simulink library "casper_library_sources"  (R2021a)
settings: Solver=ode45  StartTime=0.0  StopTime=10.0  RelTol=1e-3
values from neighbouring files (symbols this model uses):
  a = [lenba, lenpa, lenta]    [bus_addsub_init.m]    (also in bus_logical_init.m; bus_maddsub_init.m; bus_mult_init.m; bus_relational_init.m)
  b = [lenbb, lenpb, lentb]    [bus_addsub_init.m]    (also in bus_logical_init.m; bus_maddsub_init.m; bus_mult_init.m; bus_relational_init.m)
libraries: xbsIndex_r4 x11172, $bdroot x2
(part 6 of 29)

== system casper_library_sources/Correlation Control Block/corr_ctrl_blk/NS 27bit/lfsr_11 ==
  " reset" : Inport
  Assert{1..31} (31 alike) : xbsIndex_r4/Assert  assert_type=on  type_source=Explicitly  gui_display_data_type=Fixed-point  arith_type=Unsigned  n_bits=1  bin_pt=0  preci_type=Single  exp_width=8  frac_width=24  assert_rate=on  rate_source=Explicitly  period=1  output_port=on  block_type=assert
      settings: infoedit=Asserts a user-defined sample rate and/or type on a signal.<P><P>Hardware notes: In hardware this block costs nothing.  block_version=10.1.3
  Concat : xbsIndex_r4/Concat  num_inputs=4  dbl_ovrd=off  block_type=concat
      settings: block_version=10.1.3
  Expression{,1..11} (12 alike) : xbsIndex_r4/Expression  expression=a ^ b  align_bp=on  en=off  latency=0  precision=Full  arith_type=Unsigned  n_bits=8  bin_pt=2  dbl_ovrd=off  block_type=expr
      settings: xl_area=[0, 0, 0, 0, 0, 0, 0]  block_version=10.1.3
  Register1 : xbsIndex_r4/Register  init=seed(3)  rst=on  en=off  dbl_ovrd=off  block_type=register
      settings: xl_area=[0, 0, 0, 0, 0, 0, 0]
  Register10 : xbsIndex_r4/Register  init=seed(11)  rst=on  en=off  dbl_ovrd=off  block_type=register
      settings: xl_area=[0, 0, 0, 0, 0, 0, 0]
  Register11 : xbsIndex_r4/Register  init=seed(12)  rst=on  en=off  dbl_ovrd=off  block_type=register
      settings: xl_area=[0, 0, 0, 0, 0, 0, 0]
  Register12 : xbsIndex_r4/Register  init=seed(13)  rst=on  en=off  dbl_ovrd=off  block_type=register
      settings: xl_area=[0, 0, 0, 0, 0, 0, 0]
  Register13 : xbsIndex_r4/Register  init=seed(14)  rst=on  en=off  dbl_ovrd=off  block_type=register
      settings: xl_area=[0, 0, 0, 0, 0, 0, 0]
  Register14 : xbsIndex_r4/Register  init=seed(15)  rst=on  en=off  dbl_ovrd=off  block_type=register
      settings: xl_area=[0, 0, 0, 0, 0, 0, 0]
  Register15 : xbsIndex_r4/Register  init=seed(16)  rst=on  en=off  dbl_ovrd=off  block_type=register
      settings: xl_area=[0, 0, 0, 0, 0, 0, 0]
  Register16 : xbsIndex_r4/Register  init=seed(17)  rst=on  en=off  dbl_ovrd=off  block_type=register
      settings: xl_area=[0, 0, 0, 0, 0, 0, 0]
  Register{17,19..27} (10 alike) : xbsIndex_r4/Register  init=seed(18)  rst=on  en=off  dbl_ovrd=off  block_type=register
      settings: xl_area=[0, 0, 0, 0, 0, 0, 0]
  Register18 : xbsIndex_r4/Register  init=seed(1)  rst=on  en=off  dbl_ovrd=off  block_type=register
      settings: xl_area=[0, 0, 0, 0, 0, 0, 0]
  Register2 : xbsIndex_r4/Register  init=seed(2)  rst=on  en=off  dbl_ovrd=off  block_type=register
      settings: xl_area=[0, 0, 0, 0, 0, 0, 0]
  Register3 : xbsIndex_r4/Register  init=seed(4)  rst=on  en=off  dbl_ovrd=off  block_type=register
      settings: xl_area=[0, 0, 0, 0, 0, 0, 0]
  Register4 : xbsIndex_r4/Register  init=seed(5)  rst=on  en=off  dbl_ovrd=off  block_type=register
      settings: xl_area=[0, 0, 0, 0, 0, 0, 0]
  Register5 : xbsIndex_r4/Register  init=seed(6)  rst=on  en=off  dbl_ovrd=off  block_type=register
      settings: xl_area=[0, 0, 0, 0, 0, 0, 0]
  Register6 : xbsIndex_r4/Register  init=seed(7)  rst=on  en=off  dbl_ovrd=off  block_type=register
      settings: xl_area=[0, 0, 0, 0, 0, 0, 0]
  Register7 : xbsIndex_r4/Register  init=seed(8)  rst=on  en=off  dbl_ovrd=off  block_type=register
      settings: xl_area=[0, 0, 0, 0, 0, 0, 0]
  Register8 : xbsIndex_r4/Register  init=seed(9)  rst=on  en=off  dbl_ovrd=off  block_type=register
      settings: xl_area=[0, 0, 0, 0, 0, 0, 0]
  Register9 : xbsIndex_r4/Register  init=seed(10)  rst=on  en=off  dbl_ovrd=off  block_type=register
      settings: xl_area=[0, 0, 0, 0, 0, 0, 0]
  Out1 : Outport  VectorParamsAs1DForOutWhenUnconnected=off
  wires:
  Register27/1 -> Assert31/1
  [a3] -> Register27/1
  [reset] -> Register27/2
  Assert31/1 -> [q26]
  Register26/1 -> Assert30/1
  [a2] -> Register26/1
  [reset] -> Register26/2
  Assert30/1 -> [q25]
  Register25/1 -> Assert29/1
  [a1] -> Register25/1
  [reset] -> Register25/2
  Assert29/1 -> [q24]
  Register24/1 -> Assert28/1
  [a0] -> Register24/1
  [reset] -> Register24/2
  Assert28/1 -> [q23]
  Register23/1 -> Assert27/1
  [q26] -> Register23/1
  [reset] -> Register23/2
  Assert27/1 -> [q22]
  Register22/1 -> Assert26/1
  [q25] -> Register22/1
  [reset] -> Register22/2
  Assert26/1 -> [q21]
  Register21/1 -> Assert25/1
  [q24] -> Register21/1
  [reset] -> Register21/2
  Assert25/1 -> [q20]
  Register20/1 -> Assert24/1
  [q23] -> Register20/1
  [reset] -> Register20/2
  Assert24/1 -> [q19]
  Register19/1 -> Assert23/1
  [q22] -> Register19/1
  [reset] -> Register19/2
  Assert23/1 -> [q18]
  Register18/1 -> Assert18/1
  [q4] -> Register18/1
  [reset] -> Register18/2
  Assert18/1 -> [q0]
  [q5] -> Expression7/1
  [a0] -> Concat/4
  [a1] -> Concat/3
  [a2] -> Concat/2
  [a3] -> Concat/1
  Expression11/1 -> Assert22/1
  Expression8/1 -> Assert21/1
  Expression5/1 -> Assert20/1
  Expression2/1 -> Assert19/1
  Concat/1 -> Out1/1
  Expression10/1 -> Expression11/2
  Expression9/1 -> Expression11/1
  [q19] -> Expression10/2
  [q6] -> Expression10/1
  [q4] -> Expression9/2
  [q3] -> Expression9/1
  [q18] -> Expression7/2
  [q3] -> Expression6/2
  [q2] -> Expression6/1
  [q17] -> Expression4/2
  [q4] -> Expression4/1
  [q2] -> Expression3/2
  [q1] -> Expression3/1
  [q16] -> Expression1/2
  [q3] -> Expression1/1
  [q1] -> Expression/2
  [q0] -> Expression/1
  Register17/1 -> Assert17/1
  Register16/1 -> Assert16/1
  Register15/1 -> Assert15/1
  Register14/1 -> Assert14/1
  Register13/1 -> Assert13/1
  Register12/1 -> Assert12/1
  Register11/1 -> Assert11/1
  Register10/1 -> Assert10/1
  Register9/1 -> Assert9/1
  Register8/1 -> Assert8/1
  Register7/1 -> Assert7/1
  Register6/1 -> Assert6/1
  Register5/1 -> Assert5/1
  Register4/1 -> Assert4/1
  Register3/1 -> Assert3/1
  Register1/1 -> Assert2/1
  Register2/1 -> Assert1/1
  [q21] -> Register17/1
  [q20] -> Register16/1
  [q19] -> Register15/1
  [q18] -> Register14/1
  [q17] -> Register13/1
  [q16] -> Register12/1
  [q15] -> Register11/1
  [q14] -> Register10/1
  [q13] -> Register9/1
  [q12] -> Register8/1
  [q11] -> Register7/1
  [q10] -> Register6/1
  [q9] -> Register5/1
  [q8] -> Register4/1
  [q7] -> Register3/1
  [q6] -> Register1/1
  [q5] -> Register2/1
  [reset] -> Register17/2
  [reset] -> Register16/2
  [reset] -> Register15/2
  [reset] -> Register14/2
  [reset] -> Register13/2
  [reset] -> Register12/2
  [reset] -> Register11/2
  [reset] -> Register10/2
  [reset] -> Register9/2
  [reset] -> Register8/2
  [reset] -> Register7/2
  [reset] -> Register6/2
  [reset] -> Register5/2
  [reset] -> Register4/2
  [reset] -> Register3/2
  [reset] -> Register1/2
  [reset] -> Register2/2
  " reset"/1 -> [reset]
  Expression7/1 -> Expression8/2
  Expression6/1 -> Expression8/1
  Expression4/1 -> Expression5/2
  Expression3/1 -> Expression5/1
  Expression1/1 -> Expression2/2
  Expression/1 -> Expression2/1
  Assert1/1 -> [q1]
  Assert2/1 -> [q2]
  Assert3/1 -> [q3]
  Assert4/1 -> [q4]
  Assert5/1 -> [q5]
  Assert6/1 -> [q6]
  Assert7/1 -> [q7]
  Assert8/1 -> [q8]
  Assert9/1 -> [q9]
  Assert10/1 -> [q10]
  Assert11/1 -> [q11]
  Assert12/1 -> [q12]
  Assert13/1 -> [q13]
  Assert14/1 -> [q14]
  Assert15/1 -> [q15]
  Assert16/1 -> [q16]
  Assert17/1 -> [q17]
  Assert19/1 -> [a0]
  Assert20/1 -> [a1]
  Assert21/1 -> [a2]
  Assert22/1 -> [a3]

== system casper_library_sources/Correlation Control Block/corr_ctrl_blk/NS 27bit/lfsr_12 ==
  " reset" : Inport
  Assert{1..31} (31 alike) : xbsIndex_r4/Assert  assert_type=on  type_source=Explicitly  gui_display_data_type=Fixed-point  arith_type=Unsigned  n_bits=1  bin_pt=0  preci_type=Single  exp_width=8  frac_width=24  assert_rate=on  rate_source=Explicitly  period=1  output_port=on  block_type=assert
      settings: infoedit=Asserts a user-defined sample rate and/or type on a signal.<P><P>Hardware notes: In hardware this block costs nothing.  block_version=10.1.3
  Concat : xbsIndex_r4/Concat  num_inputs=4  dbl_ovrd=off  block_type=concat
      settings: block_version=10.1.3
  Expression{,1..11} (12 alike) : xbsIndex_r4/Expression  expression=a ^ b  align_bp=on  en=off  latency=0  precision=Full  arith_type=Unsigned  n_bits=8  bin_pt=2  dbl_ovrd=off  block_type=expr
      settings: xl_area=[0, 0, 0, 0, 0, 0, 0]  block_version=10.1.3
  Register1 : xbsIndex_r4/Register  init=seed(3)  rst=on  en=off  dbl_ovrd=off  block_type=register
      settings: xl_area=[0, 0, 0, 0, 0, 0, 0]
  Register10 : xbsIndex_r4/Register  init=seed(11)  rst=on  en=off  dbl_ovrd=off  block_type=register
      settings: xl_area=[0, 0, 0, 0, 0, 0, 0]
  Register11 : xbsIndex_r4/Register  init=seed(12)  rst=on  en=off  dbl_ovrd=off  block_type=register
      settings: xl_area=[0, 0, 0, 0, 0, 0, 0]
  Register12 : xbsIndex_r4/Register  init=seed(13)  rst=on  en=off  dbl_ovrd=off  block_type=register
      settings: xl_area=[0, 0, 0, 0, 0, 0, 0]
  Register13 : xbsIndex_r4/Register  init=seed(14)  rst=on  en=off  dbl_ovrd=off  block_type=register
      settings: xl_area=[0, 0, 0, 0, 0, 0, 0]
  Register14 : xbsIndex_r4/Register  init=seed(15)  rst=on  en=off  dbl_ovrd=off  block_type=register
      settings: xl_area=[0, 0, 0, 0, 0, 0, 0]
  Register15 : xbsIndex_r4/Register  init=seed(16)  rst=on  en=off  dbl_ovrd=off  block_type=register
      settings: xl_area=[0, 0, 0, 0, 0, 0, 0]
  Register16 : xbsIndex_r4/Register  init=seed(17)  rst=on  en=off  dbl_ovrd=off  block_type=register
      settings: xl_area=[0, 0, 0, 0, 0, 0, 0]
  Register{17,19..27} (10 alike) : xbsIndex_r4/Register  init=seed(18)  rst=on  en=off  dbl_ovrd=off  block_type=register
      settings: xl_area=[0, 0, 0, 0, 0, 0, 0]
  Register18 : xbsIndex_r4/Register  init=seed(1)  rst=on  en=off  dbl_ovrd=off  block_type=register
      settings: xl_area=[0, 0, 0, 0, 0, 0, 0]
  Register2 : xbsIndex_r4/Register  init=seed(2)  rst=on  en=off  dbl_ovrd=off  block_type=register
      settings: xl_area=[0, 0, 0, 0, 0, 0, 0]
  Register3 : xbsIndex_r4/Register  init=seed(4)  rst=on  en=off  dbl_ovrd=off  block_type=register
      settings: xl_area=[0, 0, 0, 0, 0, 0, 0]
  Register4 : xbsIndex_r4/Register  init=seed(5)  rst=on  en=off  dbl_ovrd=off  block_type=register
      settings: xl_area=[0, 0, 0, 0, 0, 0, 0]
  Register5 : xbsIndex_r4/Register  init=seed(6)  rst=on  en=off  dbl_ovrd=off  block_type=register
      settings: xl_area=[0, 0, 0, 0, 0, 0, 0]
  Register6 : xbsIndex_r4/Register  init=seed(7)  rst=on  en=off  dbl_ovrd=off  block_type=register
      settings: xl_area=[0, 0, 0, 0, 0, 0, 0]
  Register7 : xbsIndex_r4/Register  init=seed(8)  rst=on  en=off  dbl_ovrd=off  block_type=register
      settings: xl_area=[0, 0, 0, 0, 0, 0, 0]
  Register8 : xbsIndex_r4/Register  init=seed(9)  rst=on  en=off  dbl_ovrd=off  block_type=register
      settings: xl_area=[0, 0, 0, 0, 0, 0, 0]
  Register9 : xbsIndex_r4/Register  init=seed(10)  rst=on  en=off  dbl_ovrd=off  block_type=register
      settings: xl_area=[0, 0, 0, 0, 0, 0, 0]
  Out1 : Outport  VectorParamsAs1DForOutWhenUnconnected=off
  wires:
  Assert22/1 -> [a3]
  Assert21/1 -> [a2]
  Assert20/1 -> [a1]
  Assert19/1 -> [a0]
  Assert17/1 -> [q17]
  Assert16/1 -> [q16]
  Assert15/1 -> [q15]
  Assert14/1 -> [q14]
  Assert13/1 -> [q13]
  Assert12/1 -> [q12]
  Assert11/1 -> [q11]
  Assert10/1 -> [q10]
  Assert9/1 -> [q9]
  Assert8/1 -> [q8]
  Assert7/1 -> [q7]
  Assert6/1 -> [q6]
  Assert5/1 -> [q5]
  Assert4/1 -> [q4]
  Assert3/1 -> [q3]
  Assert2/1 -> [q2]
  Assert1/1 -> [q1]
  Expression/1 -> Expression2/1
  Expression1/1 -> Expression2/2
  Expression3/1 -> Expression5/1
  Expression4/1 -> Expression5/2
  Expression6/1 -> Expression8/1
  Expression7/1 -> Expression8/2
  " reset"/1 -> [reset]
  [reset] -> Register2/2
  [reset] -> Register1/2
  [reset] -> Register3/2
  [reset] -> Register4/2
  [reset] -> Register5/2
  [reset] -> Register6/2
  [reset] -> Register7/2
  [reset] -> Register8/2
  [reset] -> Register9/2
  [reset] -> Register10/2
  [reset] -> Register11/2
  [reset] -> Register12/2
  [reset] -> Register13/2
  [reset] -> Register14/2
  [reset] -> Register15/2
  [reset] -> Register16/2
  [reset] -> Register17/2
  [q5] -> Register2/1
  [q6] -> Register1/1
  [q7] -> Register3/1
  [q8] -> Register4/1
  [q9] -> Register5/1
  [q10] -> Register6/1
  [q11] -> Register7/1
  [q12] -> Register8/1
  [q13] -> Register9/1
  [q14] -> Register10/1
  [q15] -> Register11/1
  [q16] -> Register12/1
  [q17] -> Register13/1
  [q18] -> Register14/1
  [q19] -> Register15/1
  [q20] -> Register16/1
  [q21] -> Register17/1
  Register2/1 -> Assert1/1
  Register1/1 -> Assert2/1
  Register3/1 -> Assert3/1
  Register4/1 -> Assert4/1
  Register5/1 -> Assert5/1
  Register6/1 -> Assert6/1
  Register7/1 -> Assert7/1
  Register8/1 -> Assert8/1
  Register9/1 -> Assert9/1
  Register10/1 -> Assert10/1
  Register11/1 -> Assert11/1
  Register12/1 -> Assert12/1
  Register13/1 -> Assert13/1
  Register14/1 -> Assert14/1
  Register15/1 -> Assert15/1
  Register16/1 -> Assert16/1
  Register17/1 -> Assert17/1
  [q0] -> Expression/1
  [q1] -> Expression/2
  [q3] -> Expression1/1
  [q16] -> Expression1/2
  [q1] -> Expression3/1
  [q2] -> Expression3/2
  [q4] -> Expression4/1
  [q17] -> Expression4/2
  [q2] -> Expression6/1
  [q3] -> Expression6/2
  [q18] -> Expression7/2
  [q3] -> Expression9/1
  [q4] -> Expression9/2
  [q6] -> Expression10/1
  [q19] -> Expression10/2
  Expression9/1 -> Expression11/1
  Expression10/1 -> Expression11/2
  Concat/1 -> Out1/1
  Expression2/1 -> Assert19/1
  Expression5/1 -> Assert20/1
  Expression8/1 -> Assert21/1
  Expression11/1 -> Assert22/1
  [a3] -> Concat/1
  [a2] -> Concat/2
  [a1] -> Concat/3
  [a0] -> Concat/4
  [q5] -> Expression7/1
  Assert18/1 -> [q0]
  [reset] -> Register18/2
  [q4] -> Register18/1
  Register18/1 -> Assert18/1
  Assert23/1 -> [q18]
  [reset] -> Register19/2
  [q22] -> Register19/1
  Register19/1 -> Assert23/1
  Assert24/1 -> [q19]
  [reset] -> Register20/2
  [q23] -> Register20/1
  Register20/1 -> Assert24/1
  Assert25/1 -> [q20]
  [reset] -> Register21/2
  [q24] -> Register21/1
  Register21/1 -> Assert25/1
  Assert26/1 -> [q21]
  [reset] -> Register22/2
  [q25] -> Register22/1
  Register22/1 -> Assert26/1
  Assert27/1 -> [q22]
  [reset] -> Register23/2
  [q26] -> Register23/1
  Register23/1 -> Assert27/1
  Assert28/1 -> [q23]
  [reset] -> Register24/2
  [a0] -> Register24/1
  Register24/1 -> Assert28/1
  Assert29/1 -> [q24]
  [reset] -> Register25/2
  [a1] -> Register25/1
  Register25/1 -> Assert29/1
  Assert30/1 -> [q25]
  [reset] -> Register26/2
  [a2] -> Register26/1
  Register26/1 -> Assert30/1
  Assert31/1 -> [q26]
  [reset] -> Register27/2
  [a3] -> Register27/1
  Register27/1 -> Assert31/1

== system casper_library_sources/Correlation Control Block/corr_ctrl_blk/NS 27bit/lfsr_13 ==
  " reset" : Inport
  Assert{1..31} (31 alike) : xbsIndex_r4/Assert  assert_type=on  type_source=Explicitly  gui_display_data_type=Fixed-point  arith_type=Unsigned  n_bits=1  bin_pt=0  preci_type=Single  exp_width=8  frac_width=24  assert_rate=on  rate_source=Explicitly  period=1  output_port=on  block_type=assert
      settings: infoedit=Asserts a user-defined sample rate and/or type on a signal.<P><P>Hardware notes: In hardware this block costs nothing.  block_version=10.1.3
  Concat : xbsIndex_r4/Concat  num_inputs=4  dbl_ovrd=off  block_type=concat
      settings: block_version=10.1.3
  Expression{,1..11} (12 alike) : xbsIndex_r4/Expression  expression=a ^ b  align_bp=on  en=off  latency=0  precision=Full  arith_type=Unsigned  n_bits=8  bin_pt=2  dbl_ovrd=off  block_type=expr
      settings: xl_area=[0, 0, 0, 0, 0, 0, 0]  block_version=10.1.3
  Register1 : xbsIndex_r4/Register  init=seed(3)  rst=on  en=off  dbl_ovrd=off  block_type=register
      settings: xl_area=[0, 0, 0, 0, 0, 0, 0]
  Register10 : xbsIndex_r4/Register  init=seed(11)  rst=on  en=off  dbl_ovrd=off  block_type=register
      settings: xl_area=[0, 0, 0, 0, 0, 0, 0]
  Register11 : xbsIndex_r4/Register  init=seed(12)  rst=on  en=off  dbl_ovrd=off  block_type=register
      settings: xl_area=[0, 0, 0, 0, 0, 0, 0]
  Register12 : xbsIndex_r4/Register  init=seed(13)  rst=on  en=off  dbl_ovrd=off  block_type=register
      settings: xl_area=[0, 0, 0, 0, 0, 0, 0]
  Register13 : xbsIndex_r4/Register  init=seed(14)  rst=on  en=off  dbl_ovrd=off  block_type=register
      settings: xl_area=[0, 0, 0, 0, 0, 0, 0]
  Register14 : xbsIndex_r4/Register  init=seed(15)  rst=on  en=off  dbl_ovrd=off  block_type=register
      settings: xl_area=[0, 0, 0, 0, 0, 0, 0]
  Register15 : xbsIndex_r4/Register  init=seed(16)  rst=on  en=off  dbl_ovrd=off  block_type=register
      settings: xl_area=[0, 0, 0, 0, 0, 0, 0]
  Register16 : xbsIndex_r4/Register  init=seed(17)  rst=on  en=off  dbl_ovrd=off  block_type=register
      settings: xl_area=[0, 0, 0, 0, 0, 0, 0]
  Register{17,19..27} (10 alike) : xbsIndex_r4/Register  init=seed(18)  rst=on  en=off  dbl_ovrd=off  block_type=register
      settings: xl_area=[0, 0, 0, 0, 0, 0, 0]
  Register18 : xbsIndex_r4/Register  init=seed(1)  rst=on  en=off  dbl_ovrd=off  block_type=register
      settings: xl_area=[0, 0, 0, 0, 0, 0, 0]
  Register2 : xbsIndex_r4/Register  init=seed(2)  rst=on  en=off  dbl_ovrd=off  block_type=register
      settings: xl_area=[0, 0, 0, 0, 0, 0, 0]
  Register3 : xbsIndex_r4/Register  init=seed(4)  rst=on  en=off  dbl_ovrd=off  block_type=register
      settings: xl_area=[0, 0, 0, 0, 0, 0, 0]
  Register4 : xbsIndex_r4/Register  init=seed(5)  rst=on  en=off  dbl_ovrd=off  block_type=register
      settings: xl_area=[0, 0, 0, 0, 0, 0, 0]
  Register5 : xbsIndex_r4/Register  init=seed(6)  rst=on  en=off  dbl_ovrd=off  block_type=register
      settings: xl_area=[0, 0, 0, 0, 0, 0, 0]
  Register6 : xbsIndex_r4/Register  init=seed(7)  rst=on  en=off  dbl_ovrd=off  block_type=register
      settings: xl_area=[0, 0, 0, 0, 0, 0, 0]
  Register7 : xbsIndex_r4/Register  init=seed(8)  rst=on  en=off  dbl_ovrd=off  block_type=register
      settings: xl_area=[0, 0, 0, 0, 0, 0, 0]
  Register8 : xbsIndex_r4/Register  init=seed(9)  rst=on  en=off  dbl_ovrd=off  block_type=register
      settings: xl_area=[0, 0, 0, 0, 0, 0, 0]
  Register9 : xbsIndex_r4/Register  init=seed(10)  rst=on  en=off  dbl_ovrd=off  block_type=register
      settings: xl_area=[0, 0, 0, 0, 0, 0, 0]
  Out1 : Outport  VectorParamsAs1DForOutWhenUnconnected=off
  wires:
  Register27/1 -> Assert31/1
  [a3] -> Register27/1
  [reset] -> Register27/2
  Assert31/1 -> [q26]
  Register26/1 -> Assert30/1
  [a2] -> Register26/1
  [reset] -> Register26/2
  Assert30/1 -> [q25]
  Register25/1 -> Assert29/1
  [a1] -> Register25/1
  [reset] -> Register25/2
  Assert29/1 -> [q24]
  Register24/1 -> Assert28/1
  [a0] -> Register24/1
  [reset] -> Register24/2
  Assert28/1 -> [q23]
  Register23/1 -> Assert27/1
  [q26] -> Register23/1
  [reset] -> Register23/2
  Assert27/1 -> [q22]
  Register22/1 -> Assert26/1
  [q25] -> Register22/1
  [reset] -> Register22/2
  Assert26/1 -> [q21]
  Register21/1 -> Assert25/1
  [q24] -> Register21/1
  [reset] -> Register21/2
  Assert25/1 -> [q20]
  Register20/1 -> Assert24/1
  [q23] -> Register20/1
  [reset] -> Register20/2
  Assert24/1 -> [q19]
  Register19/1 -> Assert23/1
  [q22] -> Register19/1
  [reset] -> Register19/2
  Assert23/1 -> [q18]
  Register18/1 -> Assert18/1
  [q4] -> Register18/1
  [reset] -> Register18/2
  Assert18/1 -> [q0]
  [q5] -> Expression7/1
  [a0] -> Concat/4
  [a1] -> Concat/3
  [a2] -> Concat/2
  [a3] -> Concat/1
  Expression11/1 -> Assert22/1
  Expression8/1 -> Assert21/1
  Expression5/1 -> Assert20/1
  Expression2/1 -> Assert19/1
  Concat/1 -> Out1/1
  Expression10/1 -> Expression11/2
  Expression9/1 -> Expression11/1
  [q19] -> Expression10/2
  [q6] -> Expression10/1
  [q4] -> Expression9/2
  [q3] -> Expression9/1
  [q18] -> Expression7/2
  [q3] -> Expression6/2
  [q2] -> Expression6/1
  [q17] -> Expression4/2
  [q4] -> Expression4/1
  [q2] -> Expression3/2
  [q1] -> Expression3/1
  [q16] -> Expression1/2
  [q3] -> Expression1/1
  [q1] -> Expression/2
  [q0] -> Expression/1
  Register17/1 -> Assert17/1
  Register16/1 -> Assert16/1
  Register15/1 -> Assert15/1
  Register14/1 -> Assert14/1
  Register13/1 -> Assert13/1
  Register12/1 -> Assert12/1
  Register11/1 -> Assert11/1
  Register10/1 -> Assert10/1
  Register9/1 -> Assert9/1
  Register8/1 -> Assert8/1
  Register7/1 -> Assert7/1
  Register6/1 -> Assert6/1
  Register5/1 -> Assert5/1
  Register4/1 -> Assert4/1
  Register3/1 -> Assert3/1
  Register1/1 -> Assert2/1
  Register2/1 -> Assert1/1
  [q21] -> Register17/1
  [q20] -> Register16/1
  [q19] -> Register15/1
  [q18] -> Register14/1
  [q17] -> Register13/1
  [q16] -> Register12/1
  [q15] -> Register11/1
  [q14] -> Register10/1
  [q13] -> Register9/1
  [q12] -> Register8/1
  [q11] -> Register7/1
  [q10] -> Register6/1
  [q9] -> Register5/1
  [q8] -> Register4/1
  [q7] -> Register3/1
  [q6] -> Register1/1
  [q5] -> Register2/1
  [reset] -> Register17/2
  [reset] -> Register16/2
  [reset] -> Register15/2
  [reset] -> Register14/2
  [reset] -> Register13/2
  [reset] -> Register12/2
  [reset] -> Register11/2
  [reset] -> Register10/2
  [reset] -> Register9/2
  [reset] -> Register8/2
  [reset] -> Register7/2
  [reset] -> Register6/2
  [reset] -> Register5/2
  [reset] -> Register4/2
  [reset] -> Register3/2
  [reset] -> Register1/2
  [reset] -> Register2/2
  " reset"/1 -> [reset]
  Expression7/1 -> Expression8/2
  Expression6/1 -> Expression8/1
  Expression4/1 -> Expression5/2
  Expression3/1 -> Expression5/1
  Expression1/1 -> Expression2/2
  Expression/1 -> Expression2/1
  Assert1/1 -> [q1]
  Assert2/1 -> [q2]
  Assert3/1 -> [q3]
  Assert4/1 -> [q4]
  Assert5/1 -> [q5]
  Assert6/1 -> [q6]
  Assert7/1 -> [q7]
  Assert8/1 -> [q8]
  Assert9/1 -> [q9]
  Assert10/1 -> [q10]
  Assert11/1 -> [q11]
  Assert12/1 -> [q12]
  Assert13/1 -> [q13]
  Assert14/1 -> [q14]
  Assert15/1 -> [q15]
  Assert16/1 -> [q16]
  Assert17/1 -> [q17]
  Assert19/1 -> [a0]
  Assert20/1 -> [a1]
  Assert21/1 -> [a2]
  Assert22/1 -> [a3]

== system casper_library_sources/Correlation Control Block/corr_ctrl_blk/NS 27bit/lfsr_14 ==
  " reset" : Inport
  Assert{1..31} (31 alike) : xbsIndex_r4/Assert  assert_type=on  type_source=Explicitly  gui_display_data_type=Fixed-point  arith_type=Unsigned  n_bits=1  bin_pt=0  preci_type=Single  exp_width=8  frac_width=24  assert_rate=on  rate_source=Explicitly  period=1  output_port=on  block_type=assert
      settings: infoedit=Asserts a user-defined sample rate and/or type on a signal.<P><P>Hardware notes: In hardware this block costs nothing.  block_version=10.1.3
  Concat : xbsIndex_r4/Concat  num_inputs=4  dbl_ovrd=off  block_type=concat
      settings: block_version=10.1.3
  Expression{,1..11} (12 alike) : xbsIndex_r4/Expression  expression=a ^ b  align_bp=on  en=off  latency=0  precision=Full  arith_type=Unsigned  n_bits=8  bin_pt=2  dbl_ovrd=off  block_type=expr
      settings: xl_area=[0, 0, 0, 0, 0, 0, 0]  block_version=10.1.3
  Register1 : xbsIndex_r4/Register  init=seed(3)  rst=on  en=off  dbl_ovrd=off  block_type=register
      settings: xl_area=[0, 0, 0, 0, 0, 0, 0]
  Register10 : xbsIndex_r4/Register  init=seed(11)  rst=on  en=off  dbl_ovrd=off  block_type=register
      settings: xl_area=[0, 0, 0, 0, 0, 0, 0]
  Register11 : xbsIndex_r4/Register  init=seed(12)  rst=on  en=off  dbl_ovrd=off  block_type=register
      settings: xl_area=[0, 0, 0, 0, 0, 0, 0]
  Register12 : xbsIndex_r4/Register  init=seed(13)  rst=on  en=off  dbl_ovrd=off  block_type=register
      settings: xl_area=[0, 0, 0, 0, 0, 0, 0]
  Register13 : xbsIndex_r4/Register  init=seed(14)  rst=on  en=off  dbl_ovrd=off  block_type=register
      settings: xl_area=[0, 0, 0, 0, 0, 0, 0]
  Register14 : xbsIndex_r4/Register  init=seed(15)  rst=on  en=off  dbl_ovrd=off  block_type=register
      settings: xl_area=[0, 0, 0, 0, 0, 0, 0]
  Register15 : xbsIndex_r4/Register  init=seed(16)  rst=on  en=off  dbl_ovrd=off  block_type=register
      settings: xl_area=[0, 0, 0, 0, 0, 0, 0]
  Register16 : xbsIndex_r4/Register  init=seed(17)  rst=on  en=off  dbl_ovrd=off  block_type=register
      settings: xl_area=[0, 0, 0, 0, 0, 0, 0]
  Register{17,19..27} (10 alike) : xbsIndex_r4/Register  init=seed(18)  rst=on  en=off  dbl_ovrd=off  block_type=register
      settings: xl_area=[0, 0, 0, 0, 0, 0, 0]
  Register18 : xbsIndex_r4/Register  init=seed(1)  rst=on  en=off  dbl_ovrd=off  block_type=register
      settings: xl_area=[0, 0, 0, 0, 0, 0, 0]
  Register2 : xbsIndex_r4/Register  init=seed(2)  rst=on  en=off  dbl_ovrd=off  block_type=register
      settings: xl_area=[0, 0, 0, 0, 0, 0, 0]
  Register3 : xbsIndex_r4/Register  init=seed(4)  rst=on  en=off  dbl_ovrd=off  block_type=register
      settings: xl_area=[0, 0, 0, 0, 0, 0, 0]
  Register4 : xbsIndex_r4/Register  init=seed(5)  rst=on  en=off  dbl_ovrd=off  block_type=register
      settings: xl_area=[0, 0, 0, 0, 0, 0, 0]
  Register5 : xbsIndex_r4/Register  init=seed(6)  rst=on  en=off  dbl_ovrd=off  block_type=register
      settings: xl_area=[0, 0, 0, 0, 0, 0, 0]
  Register6 : xbsIndex_r4/Register  init=seed(7)  rst=on  en=off  dbl_ovrd=off  block_type=register
      settings: xl_area=[0, 0, 0, 0, 0, 0, 0]
  Register7 : xbsIndex_r4/Register  init=seed(8)  rst=on  en=off  dbl_ovrd=off  block_type=register
      settings: xl_area=[0, 0, 0, 0, 0, 0, 0]
  Register8 : xbsIndex_r4/Register  init=seed(9)  rst=on  en=off  dbl_ovrd=off  block_type=register
      settings: xl_area=[0, 0, 0, 0, 0, 0, 0]
  Register9 : xbsIndex_r4/Register  init=seed(10)  rst=on  en=off  dbl_ovrd=off  block_type=register
      settings: xl_area=[0, 0, 0, 0, 0, 0, 0]
  Out1 : Outport  VectorParamsAs1DForOutWhenUnconnected=off
  wires:
  Assert22/1 -> [a3]
  Assert21/1 -> [a2]
  Assert20/1 -> [a1]
  Assert19/1 -> [a0]
  Assert17/1 -> [q17]
  Assert16/1 -> [q16]
  Assert15/1 -> [q15]
  Assert14/1 -> [q14]
  Assert13/1 -> [q13]
  Assert12/1 -> [q12]
  Assert11/1 -> [q11]
  Assert10/1 -> [q10]
  Assert9/1 -> [q9]
  Assert8/1 -> [q8]
  Assert7/1 -> [q7]
  Assert6/1 -> [q6]
  Assert5/1 -> [q5]
  Assert4/1 -> [q4]
  Assert3/1 -> [q3]
  Assert2/1 -> [q2]
  Assert1/1 -> [q1]
  Expression/1 -> Expression2/1
  Expression1/1 -> Expression2/2
  Expression3/1 -> Expression5/1
  Expression4/1 -> Expression5/2
  Expression6/1 -> Expression8/1
  Expression7/1 -> Expression8/2
  " reset"/1 -> [reset]
  [reset] -> Register2/2
  [reset] -> Register1/2
  [reset] -> Register3/2
  [reset] -> Register4/2
  [reset] -> Register5/2
  [reset] -> Register6/2
  [reset] -> Register7/2
  [reset] -> Register8/2
  [reset] -> Register9/2
  [reset] -> Register10/2
  [reset] -> Register11/2
  [reset] -> Register12/2
  [reset] -> Register13/2
  [reset] -> Register14/2
  [reset] -> Register15/2
  [reset] -> Register16/2
  [reset] -> Register17/2
  [q5] -> Register2/1
  [q6] -> Register1/1
  [q7] -> Register3/1
  [q8] -> Register4/1
  [q9] -> Register5/1
  [q10] -> Register6/1
  [q11] -> Register7/1
  [q12] -> Register8/1
  [q13] -> Register9/1
  [q14] -> Register10/1
  [q15] -> Register11/1
  [q16] -> Register12/1
  [q17] -> Register13/1
  [q18] -> Register14/1
  [q19] -> Register15/1
  [q20] -> Register16/1
  [q21] -> Register17/1
  Register2/1 -> Assert1/1
  Register1/1 -> Assert2/1
  Register3/1 -> Assert3/1
  Register4/1 -> Assert4/1
  Register5/1 -> Assert5/1
  Register6/1 -> Assert6/1
  Register7/1 -> Assert7/1
  Register8/1 -> Assert8/1
  Register9/1 -> Assert9/1
  Register10/1 -> Assert10/1
  Register11/1 -> Assert11/1
  Register12/1 -> Assert12/1
  Register13/1 -> Assert13/1
  Register14/1 -> Assert14/1
  Register15/1 -> Assert15/1
  Register16/1 -> Assert16/1
  Register17/1 -> Assert17/1
  [q0] -> Expression/1
  [q1] -> Expression/2
  [q3] -> Expression1/1
  [q16] -> Expression1/2
  [q1] -> Expression3/1
  [q2] -> Expression3/2
  [q4] -> Expression4/1
  [q17] -> Expression4/2
  [q2] -> Expression6/1
  [q3] -> Expression6/2
  [q18] -> Expression7/2
  [q3] -> Expression9/1
  [q4] -> Expression9/2
  [q6] -> Expression10/1
  [q19] -> Expression10/2
  Expression9/1 -> Expression11/1
  Expression10/1 -> Expression11/2
  Concat/1 -> Out1/1
  Expression2/1 -> Assert19/1
  Expression5/1 -> Assert20/1
  Expression8/1 -> Assert21/1
  Expression11/1 -> Assert22/1
  [a3] -> Concat/1
  [a2] -> Concat/2
  [a1] -> Concat/3
  [a0] -> Concat/4
  [q5] -> Expression7/1
  Assert18/1 -> [q0]
  [reset] -> Register18/2
  [q4] -> Register18/1
  Register18/1 -> Assert18/1
  Assert23/1 -> [q18]
  [reset] -> Register19/2
  [q22] -> Register19/1
  Register19/1 -> Assert23/1
  Assert24/1 -> [q19]
  [reset] -> Register20/2
  [q23] -> Register20/1
  Register20/1 -> Assert24/1
  Assert25/1 -> [q20]
  [reset] -> Register21/2
  [q24] -> Register21/1
  Register21/1 -> Assert25/1
  Assert26/1 -> [q21]
  [reset] -> Register22/2
  [q25] -> Register22/1
  Register22/1 -> Assert26/1
  Assert27/1 -> [q22]
  [reset] -> Register23/2
  [q26] -> Register23/1
  Register23/1 -> Assert27/1
  Assert28/1 -> [q23]
  [reset] -> Register24/2
  [a0] -> Register24/1
  Register24/1 -> Assert28/1
  Assert29/1 -> [q24]
  [reset] -> Register25/2
  [a1] -> Register25/1
  Register25/1 -> Assert29/1
  Assert30/1 -> [q25]
  [reset] -> Register26/2
  [a2] -> Register26/1
  Register26/1 -> Assert30/1
  Assert31/1 -> [q26]
  [reset] -> Register27/2
  [a3] -> Register27/1
  Register27/1 -> Assert31/1

== system casper_library_sources/Correlation Control Block/corr_ctrl_blk/NS 27bit/lfsr_2 ==
  " reset" : Inport
  Assert{1..31} (31 alike) : xbsIndex_r4/Assert  assert_type=on  type_source=Explicitly  gui_display_data_type=Fixed-point  arith_type=Unsigned  n_bits=1  bin_pt=0  preci_type=Single  exp_width=8  frac_width=24  assert_rate=on  rate_source=Explicitly  period=1  output_port=on  block_type=assert
      settings: infoedit=Asserts a user-defined sample rate and/or type on a signal.<P><P>Hardware notes: In hardware this block costs nothing.  block_version=10.1.3
  Concat : xbsIndex_r4/Concat  num_inputs=4  dbl_ovrd=off  block_type=concat
      settings: block_version=10.1.3
  Expression{,1..11} (12 alike) : xbsIndex_r4/Expression  expression=a ^ b  align_bp=on  en=off  latency=0  precision=Full  arith_type=Unsigned  n_bits=8  bin_pt=2  dbl_ovrd=off  block_type=expr
      settings: xl_area=[0, 0, 0, 0, 0, 0, 0]  block_version=10.1.3
  Register1 : xbsIndex_r4/Register  init=seed(3)  rst=on  en=off  dbl_ovrd=off  block_type=register
      settings: xl_area=[0, 0, 0, 0, 0, 0, 0]
  Register10 : xbsIndex_r4/Register  init=seed(11)  rst=on  en=off  dbl_ovrd=off  block_type=register
      settings: xl_area=[0, 0, 0, 0, 0, 0, 0]
  Register11 : xbsIndex_r4/Register  init=seed(12)  rst=on  en=off  dbl_ovrd=off  block_type=register
      settings: xl_area=[0, 0, 0, 0, 0, 0, 0]
  Register12 : xbsIndex_r4/Register  init=seed(13)  rst=on  en=off  dbl_ovrd=off  block_type=register
      settings: xl_area=[0, 0, 0, 0, 0, 0, 0]
  Register13 : xbsIndex_r4/Register  init=seed(14)  rst=on  en=off  dbl_ovrd=off  block_type=register
      settings: xl_area=[0, 0, 0, 0, 0, 0, 0]
  Register14 : xbsIndex_r4/Register  init=seed(15)  rst=on  en=off  dbl_ovrd=off  block_type=register
      settings: xl_area=[0, 0, 0, 0, 0, 0, 0]
  Register15 : xbsIndex_r4/Register  init=seed(16)  rst=on  en=off  dbl_ovrd=off  block_type=register
      settings: xl_area=[0, 0, 0, 0, 0, 0, 0]
  Register16 : xbsIndex_r4/Register  init=seed(17)  rst=on  en=off  dbl_ovrd=off  block_type=register
      settings: xl_area=[0, 0, 0, 0, 0, 0, 0]
  Register{17,19..27} (10 alike) : xbsIndex_r4/Register  init=seed(18)  rst=on  en=off  dbl_ovrd=off  block_type=register
      settings: xl_area=[0, 0, 0, 0, 0, 0, 0]
  Register18 : xbsIndex_r4/Register  init=seed(1)  rst=on  en=off  dbl_ovrd=off  block_type=register
      settings: xl_area=[0, 0, 0, 0, 0, 0, 0]
  Register2 : xbsIndex_r4/Register  init=seed(2)  rst=on  en=off  dbl_ovrd=off  block_type=register
      settings: xl_area=[0, 0, 0, 0, 0, 0, 0]
  Register3 : xbsIndex_r4/Register  init=seed(4)  rst=on  en=off  dbl_ovrd=off  block_type=register
      settings: xl_area=[0, 0, 0, 0, 0, 0, 0]
  Register4 : xbsIndex_r4/Register  init=seed(5)  rst=on  en=off  dbl_ovrd=off  block_type=register
      settings: xl_area=[0, 0, 0, 0, 0, 0, 0]
  Register5 : xbsIndex_r4/Register  init=seed(6)  rst=on  en=off  dbl_ovrd=off  block_type=register
      settings: xl_area=[0, 0, 0, 0, 0, 0, 0]
  Register6 : xbsIndex_r4/Register  init=seed(7)  rst=on  en=off  dbl_ovrd=off  block_type=register
      settings: xl_area=[0, 0, 0, 0, 0, 0, 0]
  Register7 : xbsIndex_r4/Register  init=seed(8)  rst=on  en=off  dbl_ovrd=off  block_type=register
      settings: xl_area=[0, 0, 0, 0, 0, 0, 0]
  Register8 : xbsIndex_r4/Register  init=seed(9)  rst=on  en=off  dbl_ovrd=off  block_type=register
      settings: xl_area=[0, 0, 0, 0, 0, 0, 0]
  Register9 : xbsIndex_r4/Register  init=seed(10)  rst=on  en=off  dbl_ovrd=off  block_type=register
      settings: xl_area=[0, 0, 0, 0, 0, 0, 0]
  Out1 : Outport  VectorParamsAs1DForOutWhenUnconnected=off
  wires:
  Assert22/1 -> [a3]
  Assert21/1 -> [a2]
  Assert20/1 -> [a1]
  Assert19/1 -> [a0]
  Assert17/1 -> [q17]
  Assert16/1 -> [q16]
  Assert15/1 -> [q15]
  Assert14/1 -> [q14]
  Assert13/1 -> [q13]
  Assert12/1 -> [q12]
  Assert11/1 -> [q11]
  Assert10/1 -> [q10]
  Assert9/1 -> [q9]
  Assert8/1 -> [q8]
  Assert7/1 -> [q7]
  Assert6/1 -> [q6]
  Assert5/1 -> [q5]
  Assert4/1 -> [q4]
  Assert3/1 -> [q3]
  Assert2/1 -> [q2]
  Assert1/1 -> [q1]
  Expression/1 -> Expression2/1
  Expression1/1 -> Expression2/2
  Expression3/1 -> Expression5/1
  Expression4/1 -> Expression5/2
  Expression6/1 -> Expression8/1
  Expression7/1 -> Expression8/2
  " reset"/1 -> [reset]
  [reset] -> Register2/2
  [reset] -> Register1/2
  [reset] -> Register3/2
  [reset] -> Register4/2
  [reset] -> Register5/2
  [reset] -> Register6/2
  [reset] -> Register7/2
  [reset] -> Register8/2
  [reset] -> Register9/2
  [reset] -> Register10/2
  [reset] -> Register11/2
  [reset] -> Register12/2
  [reset] -> Register13/2
  [reset] -> Register14/2
  [reset] -> Register15/2
  [reset] -> Register16/2
  [reset] -> Register17/2
  [q5] -> Register2/1
  [q6] -> Register1/1
  [q7] -> Register3/1
  [q8] -> Register4/1
  [q9] -> Register5/1
  [q10] -> Register6/1
  [q11] -> Register7/1
  [q12] -> Register8/1
  [q13] -> Register9/1
  [q14] -> Register10/1
  [q15] -> Register11/1
  [q16] -> Register12/1
  [q17] -> Register13/1
  [q18] -> Register14/1
  [q19] -> Register15/1
  [q20] -> Register16/1
  [q21] -> Register17/1
  Register2/1 -> Assert1/1
  Register1/1 -> Assert2/1
  Register3/1 -> Assert3/1
  Register4/1 -> Assert4/1
  Register5/1 -> Assert5/1
  Register6/1 -> Assert6/1
  Register7/1 -> Assert7/1
  Register8/1 -> Assert8/1
  Register9/1 -> Assert9/1
  Register10/1 -> Assert10/1
  Register11/1 -> Assert11/1
  Register12/1 -> Assert12/1
  Register13/1 -> Assert13/1
  Register14/1 -> Assert14/1
  Register15/1 -> Assert15/1
  Register16/1 -> Assert16/1
  Register17/1 -> Assert17/1
  [q0] -> Expression/1
  [q1] -> Expression/2
  [q2] -> Expression1/1
  [q5] -> Expression1/2
  [q1] -> Expression3/1
  [q2] -> Expression3/2
  [q3] -> Expression4/1
  [q6] -> Expression4/2
  [q2] -> Expression6/1
  [q3] -> Expression6/2
  [q7] -> Expression7/2
  [q3] -> Expression9/1
  [q4] -> Expression9/2
  [q5] -> Expression10/1
  [q8] -> Expression10/2
  Expression9/1 -> Expression11/1
  Expression10/1 -> Expression11/2
  Concat/1 -> Out1/1
  Expression2/1 -> Assert19/1
  Expression5/1 -> Assert20/1
  Expression8/1 -> Assert21/1
  Expression11/1 -> Assert22/1
  [a3] -> Concat/1
  [a2] -> Concat/2
  [a1] -> Concat/3
  [a0] -> Concat/4
  [q4] -> Expression7/1
  Assert18/1 -> [q0]
  [reset] -> Register18/2
  [q4] -> Register18/1
  Register18/1 -> Assert18/1
  Assert23/1 -> [q18]
  [reset] -> Register19/2
  [q22] -> Register19/1
  Register19/1 -> Assert23/1
  Assert24/1 -> [q19]
  [reset] -> Register20/2
  [q23] -> Register20/1
  Register20/1 -> Assert24/1
  Assert25/1 -> [q20]
  [reset] -> Register21/2
  [q24] -> Register21/1
  Register21/1 -> Assert25/1
  Assert26/1 -> [q21]
  [reset] -> Register22/2
  [q25] -> Register22/1
  Register22/1 -> Assert26/1
  Assert27/1 -> [q22]
  [reset] -> Register23/2
  [q26] -> Register23/1
  Register23/1 -> Assert27/1
  Assert28/1 -> [q23]
  [reset] -> Register24/2
  [a0] -> Register24/1
  Register24/1 -> Assert28/1
  Assert29/1 -> [q24]
  [reset] -> Register25/2
  [a1] -> Register25/1
  Register25/1 -> Assert29/1
  Assert30/1 -> [q25]
  [reset] -> Register26/2
  [a2] -> Register26/1
  Register26/1 -> Assert30/1
  Assert31/1 -> [q26]
  [reset] -> Register27/2
  [a3] -> Register27/1
  Register27/1 -> Assert31/1

== system casper_library_sources/Correlation Control Block/corr_ctrl_blk/NS 27bit/lfsr_3 ==
  " reset" : Inport
  Assert{1..31} (31 alike) : xbsIndex_r4/Assert  assert_type=on  type_source=Explicitly  gui_display_data_type=Fixed-point  arith_type=Unsigned  n_bits=1  bin_pt=0  preci_type=Single  exp_width=8  frac_width=24  assert_rate=on  rate_source=Explicitly  period=1  output_port=on  block_type=assert
      settings: infoedit=Asserts a user-defined sample rate and/or type on a signal.<P><P>Hardware notes: In hardware this block costs nothing.  block_version=10.1.3
  Concat : xbsIndex_r4/Concat  num_inputs=4  dbl_ovrd=off  block_type=concat
      settings: block_version=10.1.3
  Expression{,1..11} (12 alike) : xbsIndex_r4/Expression  expression=a ^ b  align_bp=on  en=off  latency=0  precision=Full  arith_type=Unsigned  n_bits=8  bin_pt=2  dbl_ovrd=off  block_type=expr
      settings: xl_area=[0, 0, 0, 0, 0, 0, 0]  block_version=10.1.3
  Register1 : xbsIndex_r4/Register  init=seed(3)  rst=on  en=off  dbl_ovrd=off  block_type=register
      settings: xl_area=[0, 0, 0, 0, 0, 0, 0]
  Register10 : xbsIndex_r4/Register  init=seed(11)  rst=on  en=off  dbl_ovrd=off  block_type=register
      settings: xl_area=[0, 0, 0, 0, 0, 0, 0]
  Register11 : xbsIndex_r4/Register  init=seed(12)  rst=on  en=off  dbl_ovrd=off  block_type=register
      settings: xl_area=[0, 0, 0, 0, 0, 0, 0]
  Register12 : xbsIndex_r4/Register  init=seed(13)  rst=on  en=off  dbl_ovrd=off  block_type=register
      settings: xl_area=[0, 0, 0, 0, 0, 0, 0]
  Register13 : xbsIndex_r4/Register  init=seed(14)  rst=on  en=off  dbl_ovrd=off  block_type=register
      settings: xl_area=[0, 0, 0, 0, 0, 0, 0]
  Register14 : xbsIndex_r4/Register  init=seed(15)  rst=on  en=off  dbl_ovrd=off  block_type=register
      settings: xl_area=[0, 0, 0, 0, 0, 0, 0]
  Register15 : xbsIndex_r4/Register  init=seed(16)  rst=on  en=off  dbl_ovrd=off  block_type=register
      settings: xl_area=[0, 0, 0, 0, 0, 0, 0]
  Register16 : xbsIndex_r4/Register  init=seed(17)  rst=on  en=off  dbl_ovrd=off  block_type=register
      settings: xl_area=[0, 0, 0, 0, 0, 0, 0]
  Register{17,19..27} (10 alike) : xbsIndex_r4/Register  init=seed(18)  rst=on  en=off  dbl_ovrd=off  block_type=register
      settings: xl_area=[0, 0, 0, 0, 0, 0, 0]
  Register18 : xbsIndex_r4/Register  init=seed(1)  rst=on  en=off  dbl_ovrd=off  block_type=register
      settings: xl_area=[0, 0, 0, 0, 0, 0, 0]
  Register2 : xbsIndex_r4/Register  init=seed(2)  rst=on  en=off  dbl_ovrd=off  block_type=register
      settings: xl_area=[0, 0, 0, 0, 0, 0, 0]
  Register3 : xbsIndex_r4/Register  init=seed(4)  rst=on  en=off  dbl_ovrd=off  block_type=register
      settings: xl_area=[0, 0, 0, 0, 0, 0, 0]
  Register4 : xbsIndex_r4/Register  init=seed(5)  rst=on  en=off  dbl_ovrd=off  block_type=register
      settings: xl_area=[0, 0, 0, 0, 0, 0, 0]
  Register5 : xbsIndex_r4/Register  init=seed(6)  rst=on  en=off  dbl_ovrd=off  block_type=register
      settings: xl_area=[0, 0, 0, 0, 0, 0, 0]
  Register6 : xbsIndex_r4/Register  init=seed(7)  rst=on  en=off  dbl_ovrd=off  block_type=register
      settings: xl_area=[0, 0, 0, 0, 0, 0, 0]
  Register7 : xbsIndex_r4/Register  init=seed(8)  rst=on  en=off  dbl_ovrd=off  block_type=register
      settings: xl_area=[0, 0, 0, 0, 0, 0, 0]
  Register8 : xbsIndex_r4/Register  init=seed(9)  rst=on  en=off  dbl_ovrd=off  block_type=register
      settings: xl_area=[0, 0, 0, 0, 0, 0, 0]
  Register9 : xbsIndex_r4/Register  init=seed(10)  rst=on  en=off  dbl_ovrd=off  block_type=register
      settings: xl_area=[0, 0, 0, 0, 0, 0, 0]
  Out1 : Outport  VectorParamsAs1DForOutWhenUnconnected=off
  wires:
  Register27/1 -> Assert31/1
  [a3] -> Register27/1
  [reset] -> Register27/2
  Assert31/1 -> [q26]
  Register26/1 -> Assert30/1
  [a2] -> Register26/1
  [reset] -> Register26/2
  Assert30/1 -> [q25]
  Register25/1 -> Assert29/1
  [a1] -> Register25/1
  [reset] -> Register25/2
  Assert29/1 -> [q24]
  Register24/1 -> Assert28/1
  [a0] -> Register24/1
  [reset] -> Register24/2
  Assert28/1 -> [q23]
  Register23/1 -> Assert27/1
  [q26] -> Register23/1
  [reset] -> Register23/2
  Assert27/1 -> [q22]
  Register22/1 -> Assert26/1
  [q25] -> Register22/1
  [reset] -> Register22/2
  Assert26/1 -> [q21]
  Register21/1 -> Assert25/1
  [q24] -> Register21/1
  [reset] -> Register21/2
  Assert25/1 -> [q20]
  Register20/1 -> Assert24/1
  [q23] -> Register20/1
  [reset] -> Register20/2
  Assert24/1 -> [q19]
  Register19/1 -> Assert23/1
  [q22] -> Register19/1
  [reset] -> Register19/2
  Assert23/1 -> [q18]
  Register18/1 -> Assert18/1
  [q4] -> Register18/1
  [reset] -> Register18/2
  Assert18/1 -> [q0]
  [q4] -> Expression7/1
  [a0] -> Concat/4
  [a1] -> Concat/3
  [a2] -> Concat/2
  [a3] -> Concat/1
  Expression11/1 -> Assert22/1
  Expression8/1 -> Assert21/1
  Expression5/1 -> Assert20/1
  Expression2/1 -> Assert19/1
  Concat/1 -> Out1/1
  Expression10/1 -> Expression11/2
  Expression9/1 -> Expression11/1
  [q8] -> Expression10/2
  [q5] -> Expression10/1
  [q4] -> Expression9/2
  [q3] -> Expression9/1
  [q7] -> Expression7/2
  [q3] -> Expression6/2
  [q2] -> Expression6/1
  [q6] -> Expression4/2
  [q3] -> Expression4/1
  [q2] -> Expression3/2
  [q1] -> Expression3/1
  [q5] -> Expression1/2
  [q2] -> Expression1/1
  [q1] -> Expression/2
  [q0] -> Expression/1
  Register17/1 -> Assert17/1
  Register16/1 -> Assert16/1
  Register15/1 -> Assert15/1
  Register14/1 -> Assert14/1
  Register13/1 -> Assert13/1
  Register12/1 -> Assert12/1
  Register11/1 -> Assert11/1
  Register10/1 -> Assert10/1
  Register9/1 -> Assert9/1
  Register8/1 -> Assert8/1
  Register7/1 -> Assert7/1
  Register6/1 -> Assert6/1
  Register5/1 -> Assert5/1
  Register4/1 -> Assert4/1
  Register3/1 -> Assert3/1
  Register1/1 -> Assert2/1
  Register2/1 -> Assert1/1
  [q21] -> Register17/1
  [q20] -> Register16/1
  [q19] -> Register15/1
  [q18] -> Register14/1
  [q17] -> Register13/1
  [q16] -> Register12/1
  [q15] -> Register11/1
  [q14] -> Register10/1
  [q13] -> Register9/1
  [q12] -> Register8/1
  [q11] -> Register7/1
  [q10] -> Register6/1
  [q9] -> Register5/1
  [q8] -> Register4/1
  [q7] -> Register3/1
  [q6] -> Register1/1
  [q5] -> Register2/1
  [reset] -> Register17/2
  [reset] -> Register16/2
  [reset] -> Register15/2
  [reset] -> Register14/2
  [reset] -> Register13/2
  [reset] -> Register12/2
  [reset] -> Register11/2
  [reset] -> Register10/2
  [reset] -> Register9/2
  [reset] -> Register8/2
  [reset] -> Register7/2
  [reset] -> Register6/2
  [reset] -> Register5/2
  [reset] -> Register4/2
  [reset] -> Register3/2
  [reset] -> Register1/2
  [reset] -> Register2/2
  " reset"/1 -> [reset]
  Expression7/1 -> Expression8/2
  Expression6/1 -> Expression8/1
  Expression4/1 -> Expression5/2
  Expression3/1 -> Expression5/1
  Expression1/1 -> Expression2/2
  Expression/1 -> Expression2/1
  Assert1/1 -> [q1]
  Assert2/1 -> [q2]
  Assert3/1 -> [q3]
  Assert4/1 -> [q4]
  Assert5/1 -> [q5]
  Assert6/1 -> [q6]
  Assert7/1 -> [q7]
  Assert8/1 -> [q8]
  Assert9/1 -> [q9]
  Assert10/1 -> [q10]
  Assert11/1 -> [q11]
  Assert12/1 -> [q12]
  Assert13/1 -> [q13]
  Assert14/1 -> [q14]
  Assert15/1 -> [q15]
  Assert16/1 -> [q16]
  Assert17/1 -> [q17]
  Assert19/1 -> [a0]
  Assert20/1 -> [a1]
  Assert21/1 -> [a2]
  Assert22/1 -> [a3]
